simulink model "inv_im_param"  (R2026b)
settings: Solver=ode23tb  StopTime=param.sim.simlength  FixedStep=tc  MaxStep=param.glb_time.tc
values from neighbouring files (symbols this model uses):
  param = add_template_extras(param, options)    [init_model.m]
undefined symbols (not defined in the file or in its folder): magnitude
libraries: fl_lib x30, nesl_utility x13, lithium_ion_battery x1, induction_machine x1, dclink_with_center_tap x1, dead_time_generator_cmos_simulink x1, three_phase_pwm_modulator x1, three_phase_inverter_ideal_switch_based_model x1, three_phase_inverter_igbt_advanced_thermal_model x1, three_phase_inverter_mosfet_based_with_thermal_model x1, threephase_inductor_lib x1, simple_flexible_shaft x1
(part 2 of 3)

== system inv_im_param/inv_im_mod1/inverter/inverter/sv_pwm ==
  gate_cmds_uvw : Inport
  Bus Selector2 : BusSelector  OutputSignals=du(k),dv(k),dw(k)
  Constant1 : Constant  Value=param.inv.behav.pwm_phase_shift_mod1
  modulator1 : Subsystem
  td2tc_1 : TransferFcn  Denominator=[param.glb_time.tc 1]
  td2tc_2 : TransferFcn  Denominator=[param.glb_time.tc 1]
  td2tc_3 : TransferFcn  Denominator=[param.glb_time.tc 1]
  gate_cmds : Outport
  wires:
  modulator1/1(gate_cmds) -> gate_cmds/1
  Constant1/1 -> modulator1/4(phase)
  Bus Selector2/1 -> td2tc_1/1  "<du(k)>"
  Bus Selector2/2 -> td2tc_2/1  "<dv(k)>"
  Bus Selector2/3 -> td2tc_3/1  "<dw(k)>"
  gate_cmds_uvw/1 -> Bus Selector2/1
  td2tc_1/1 -> modulator1/1(u)  "du(t)"
  td2tc_3/1 -> modulator1/3(w)  "dw(t)"
  td2tc_2/1 -> modulator1/2(v)  "dv(t)"

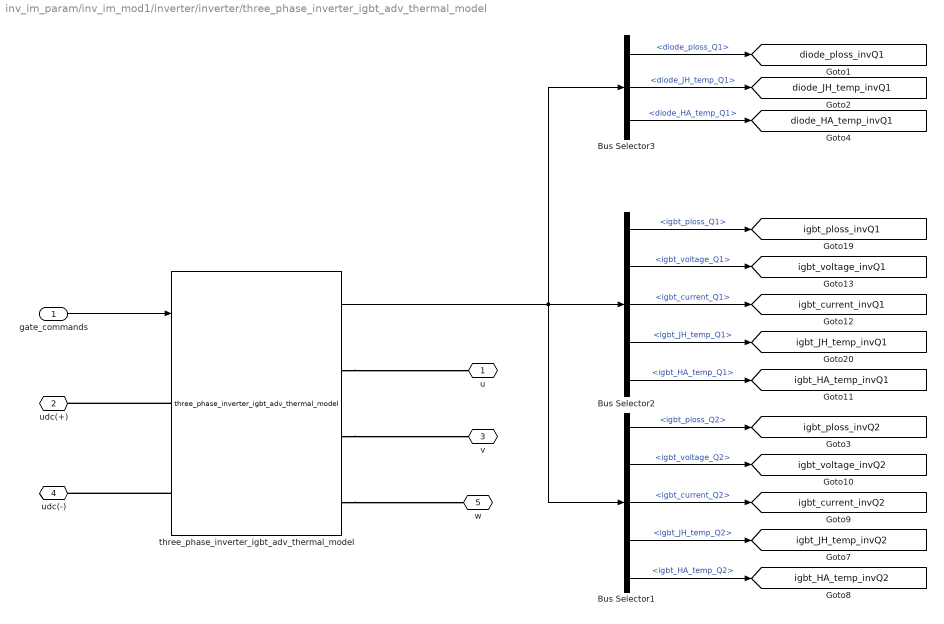
== system inv_im_param/inv_im_mod1/inverter/inverter/three_phase_inverter_igbt_adv_thermal_model ==
  gate_commands : Inport
  Bus Selector1 : BusSelector  OutputSignals=module_1.igbt_ploss_Q2,module_1.igbt_voltage_Q2,module_1.igbt_current_Q2,module_1.igbt_JH_temp_Q2,module_1.igbt_HA_temp_Q2
  Bus Selector2 : BusSelector  OutputSignals=module_1.igbt_ploss_Q1,module_1.igbt_voltage_Q1,module_1.igbt_current_Q1,module_1.igbt_JH_temp_Q1,module_1.igbt_HA_temp_Q1
  Bus Selector3 : BusSelector  OutputSignals=module_1.diode_ploss_Q1,module_1.diode_JH_temp_Q1,module_1.diode_HA_temp_Q1
  three_phase_inverter_igbt_adv_thermal_model : three_phase_inverter_igbt_advanced_thermal_model/three_phase_inverter_igbt_adv_thermal_model  mass_heatsink_m=param.thermal.weight  specific_heat_m=param.thermal.cp_al  rth_switch_HA_m=param.thermal.Rth_switch_HA  rth_switch_JH_m=param.inv.igbt.Rth_switch_JH  rth_diode_HA_m=param.thermal.Rth_diode_HA  rth_diode_JH_m=param.inv.igbt.Rth_diode_JH  Rce_on_m=param.inv.igbt.Rce_on  Vce_sat_m=param.inv.igbt.Vce_sat  Vth_m=param.inv.igbt.Vth  Eon_m=param.inv.igbt.Eon  Eoff_m=param.inv.igbt.Eoff  Erec_m=param.inv.igbt.Erec  Irr_m=param.inv.igbt.Irr  Voff_sw_loss_m=param.inv.igbt.Voff_sw_losses  Ion_sw_loss_m=param.inv.igbt.Ion_sw_losses  Vdon_diode_m=param.inv.igbt.Vdon_diode  Rdon_diode_m=param.inv.igbt.Rdon_diode  Csnubber_m=param.inv.igbt.Csnubber  Rsnubber_m=param.inv.igbt.Rsnubber  JunctionTermalMass_m=param.inv.igbt.JunctionTermalMass  Tambient_m=param.thermal.Tambient  DThs_init_m=param.thermal.DThs_init  Lstray_module_m=param.inv.igbt.Lstray_module  Cies_m=param.inv.igbt.Cies  tc_m=param.glb_time.tc
  u : PMIOPort  Side=Right
  udc(+) : PMIOPort  Port=2  Side=Left
  v : PMIOPort  Port=3  Side=Right
  udc(-) : PMIOPort  Port=4  Side=Left
  w : PMIOPort  Port=5  Side=Right
  tag scope: diode_HA_temp_invQ1=global, diode_JH_temp_invQ1=global, diode_ploss_invQ1=global, igbt_HA_temp_invQ1=global, igbt_HA_temp_invQ2=global, igbt_JH_temp_invQ1=global, igbt_JH_temp_invQ2=global, igbt_current_invQ1=global, igbt_current_invQ2=global, igbt_ploss_invQ1=global, igbt_ploss_invQ2=global, igbt_voltage_invQ1=global, igbt_voltage_invQ2=global
  wires:
  Bus Selector1/4 -> [igbt_JH_temp_invQ2]  "<igbt_JH_temp_Q2>"
  three_phase_inverter_igbt_adv_thermal_model/1 -> Bus Selector3/1, Bus Selector1/1, Bus Selector2/1
  Bus Selector1/2 -> [igbt_voltage_invQ2]  "<igbt_voltage_Q2>"
  Bus Selector1/3 -> [igbt_current_invQ2]  "<igbt_current_Q2>"
  Bus Selector1/5 -> [igbt_HA_temp_invQ2]  "<igbt_HA_temp_Q2>"
  Bus Selector2/2 -> [igbt_voltage_invQ1]  "<igbt_voltage_Q1>"
  Bus Selector2/1 -> [igbt_ploss_invQ1]  "<igbt_ploss_Q1>"
  Bus Selector2/3 -> [igbt_current_invQ1]  "<igbt_current_Q1>"
  Bus Selector1/1 -> [igbt_ploss_invQ2]  "<igbt_ploss_Q2>"
  gate_commands/1 -> three_phase_inverter_igbt_adv_thermal_model/1
  Bus Selector3/1 -> [diode_ploss_invQ1]  "<diode_ploss_Q1>"
  Bus Selector3/2 -> [diode_JH_temp_invQ1]  "<diode_JH_temp_Q1>"
  Bus Selector3/3 -> [diode_HA_temp_invQ1]  "<diode_HA_temp_Q1>"
  Bus Selector2/4 -> [igbt_JH_temp_invQ1]  "<igbt_JH_temp_Q1>"
  Bus Selector2/5 -> [igbt_HA_temp_invQ1]  "<igbt_HA_temp_Q1>"
  connections:
  three_phase_inverter_igbt_adv_thermal_model/LConn2 -- udc(-)/RConn1
  three_phase_inverter_igbt_adv_thermal_model/RConn1 -- u/RConn1
  three_phase_inverter_igbt_adv_thermal_model/RConn2 -- v/RConn1
  three_phase_inverter_igbt_adv_thermal_model/LConn1 -- udc(+)/RConn1
  three_phase_inverter_igbt_adv_thermal_model/RConn3 -- w/RConn1

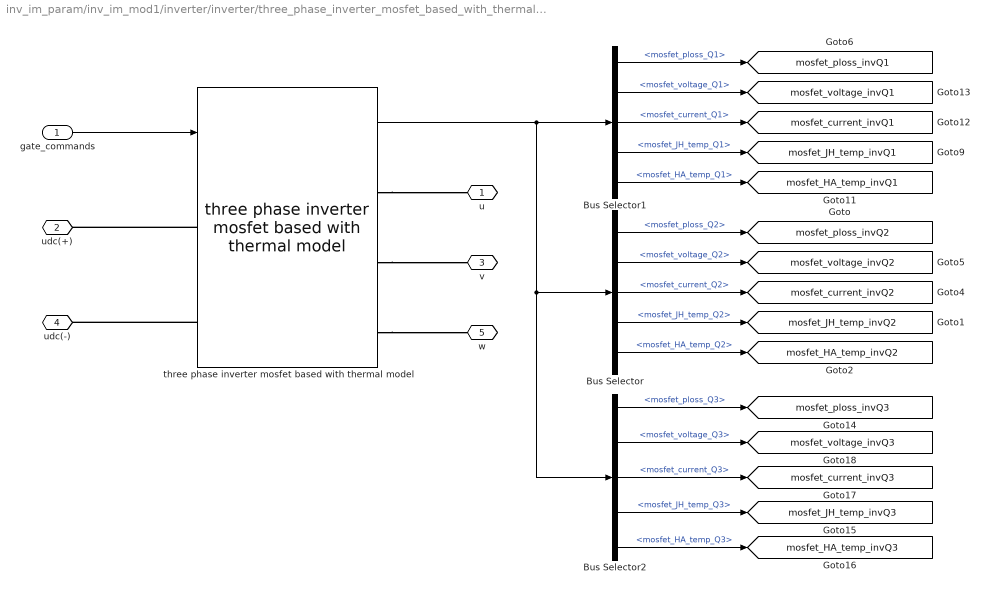
== system inv_im_param/inv_im_mod1/inverter/inverter/three_phase_inverter_mosfet_based_with_thermal_model ==
  gate_commands : Inport
  Bus Selector : BusSelector  OutputSignals=mosfet_ploss_Q2,mosfet_voltage_Q2,mosfet_current_Q2,mosfet_JH_temp_Q2,mosfet_HA_temp_Q2
  Bus Selector1 : BusSelector  OutputSignals=mosfet_ploss_Q1,mosfet_voltage_Q1,mosfet_current_Q1,mosfet_JH_temp_Q1,mosfet_HA_temp_Q1
  Bus Selector2 : BusSelector  OutputSignals=mosfet_ploss_Q3,mosfet_voltage_Q3,mosfet_current_Q3,mosfet_JH_temp_Q3,mosfet_HA_temp_Q3
  three phase inverter mosfet based with thermal model : three_phase_inverter_mosfet_based_with_thermal_model/three phase inverter mosfet based with thermal model  mass_heatsink_m=param.thermal.weight  specific_heat_m=param.thermal.cp_al  rth_mosfet_HA_m=param.thermal.Rth_diode_HA  rth_mosfet_JH_m=param.inv.mosfet.Rth_mosfet_JH  Rds_on_m=param.inv.mosfet.Rds_on  Vth_m=param.inv.mosfet.Vth  Eon_m=param.inv.mosfet.Eon  Eoff_m=param.inv.mosfet.Eoff  Voff_sw_loss_m=param.inv.mosfet.Voff_sw_losses  Ion_sw_loss_m=param.inv.mosfet.Ion_sw_losses  Vdon_diode_m=param.inv.mosfet.Vdon_diode  Rdon_diode_m=param.inv.mosfet.Rdon_diode  JunctionTermalMass_m=param.inv.mosfet.JunctionTermalMass  Tambient_m=param.thermal.Tambient  DThs_init_m=param.thermal.DThs_init
  u : PMIOPort  Side=Right
  udc(+) : PMIOPort  Port=2  Side=Left
  v : PMIOPort  Port=3  Side=Right
  udc(-) : PMIOPort  Port=4  Side=Left
  w : PMIOPort  Port=5  Side=Right
  tag scope: mosfet_HA_temp_invQ1=global, mosfet_HA_temp_invQ2=global, mosfet_HA_temp_invQ3=global, mosfet_JH_temp_invQ1=global, mosfet_JH_temp_invQ2=global, mosfet_JH_temp_invQ3=global, mosfet_current_invQ1=global, mosfet_current_invQ2=global, mosfet_current_invQ3=global, mosfet_ploss_invQ1=global, mosfet_ploss_invQ2=global, mosfet_ploss_invQ3=global, mosfet_voltage_invQ1=global, mosfet_voltage_invQ2=global, mosfet_voltage_invQ3=global
  wires:
  gate_commands/1 -> three phase inverter mosfet based with thermal model/1
  three phase inverter mosfet based with thermal model/1 -> Bus Selector/1, Bus Selector2/1, Bus Selector1/1
  Bus Selector2/1 -> [mosfet_ploss_invQ3]  "<mosfet_ploss_Q3>"
  Bus Selector2/2 -> [mosfet_voltage_invQ3]  "<mosfet_voltage_Q3>"
  Bus Selector2/3 -> [mosfet_current_invQ3]  "<mosfet_current_Q3>"
  Bus Selector2/5 -> [mosfet_HA_temp_invQ3]  "<mosfet_HA_temp_Q3>"
  Bus Selector2/4 -> [mosfet_JH_temp_invQ3]  "<mosfet_JH_temp_Q3>"
  Bus Selector/1 -> [mosfet_ploss_invQ2]  "<mosfet_ploss_Q2>"
  Bus Selector/2 -> [mosfet_voltage_invQ2]  "<mosfet_voltage_Q2>"
  Bus Selector/3 -> [mosfet_current_invQ2]  "<mosfet_current_Q2>"
  Bus Selector/4 -> [mosfet_JH_temp_invQ2]  "<mosfet_JH_temp_Q2>"
  Bus Selector/5 -> [mosfet_HA_temp_invQ2]  "<mosfet_HA_temp_Q2>"
  Bus Selector1/1 -> [mosfet_ploss_invQ1]  "<mosfet_ploss_Q1>"
  Bus Selector1/2 -> [mosfet_voltage_invQ1]  "<mosfet_voltage_Q1>"
  Bus Selector1/3 -> [mosfet_current_invQ1]  "<mosfet_current_Q1>"
  Bus Selector1/4 -> [mosfet_JH_temp_invQ1]  "<mosfet_JH_temp_Q1>"
  Bus Selector1/5 -> [mosfet_HA_temp_invQ1]  "<mosfet_HA_temp_Q1>"
  connections:
  three phase inverter mosfet based with thermal model/RConn3 -- w/RConn1
  three phase inverter mosfet based with thermal model/RConn2 -- v/RConn1
  three phase inverter mosfet based with thermal model/LConn1 -- udc(+)/RConn1
  three phase inverter mosfet based with thermal model/LConn2 -- udc(-)/RConn1
  three phase inverter mosfet based with thermal model/RConn1 -- u/RConn1

== system inv_im_param/inv_im_mod1/inverter_ctrl/im_control/Speed control ==
  rotor speed : Inport
  rotor speed ref : Inport  Port=2
  1/Ti : Gain  Gain=param.im.ctrl.kp_w  SaturateOnIntegerOverflow=on  OutDataTypeStr=Inherit: Same as input  ParamDataTypeStr=Inherit: Same as input
  Saturation : Saturate  UpperLimit=param.im.ctrl.iq_lim  LowerLimit=-param.im.ctrl.iq_lim
  Sum1 : Sum  Inputs=+++  SaturateOnIntegerOverflow=on
  Sum2 : Sum  Inputs=-+  SaturateOnIntegerOverflow=on
  Sum3 : Sum  Inputs=-+  SaturateOnIntegerOverflow=on
  Unit Delay4 : UnitDelay  SampleTime=-1
  kp : Gain  Gain=param.im.ctrl.ki_w*param.glb_time.ts_inv  SaturateOnIntegerOverflow=on  OutDataTypeStr=Inherit: Same as input  ParamDataTypeStr=Inherit: Same as input
  speed_tracking : Scope  NumInputPorts=3
      settings: ActiveDisplayYMinimum=-2.4020999013359527  ActiveDisplayYMaximum=1.8224555445928836  DataLoggingVariableName=ScopeData12
  torque_ref : Outport
  wires:
  1/Ti/1 -> Sum1/1, Sum3/1
  kp/1 -> Sum1/2
  Sum3/1 -> Unit Delay4/1
  Unit Delay4/1 -> Sum1/3
  rotor speed ref/1 -> speed_tracking/1, Sum2/2
  rotor speed/1 -> Sum2/1, speed_tracking/2
  Sum2/1 -> kp/1, 1/Ti/1
  Sum1/1 -> Saturation/1
  Saturation/1 -> torque_ref/1, speed_tracking/3, Sum3/2

== system inv_im_param/inv_im_mod1/inverter_ctrl/im_control/current_ctrl ==
  torque_ref : Inport
  Bus Creator1 : BusCreator  Inputs=2
  current_ctrl : Subsystem
  is uvw2xy : Subsystem
  rotor_flux_estimators : Subsystem
  us xy2alphabeta : Subsystem
  us xy2dq : Subsystem
  uvw2dq : Subsystem
  uab : Outport  VectorParamsAs1DForOutWhenUnconnected=off
  wires:
  [ubeta_pu_mod1] -> Bus Creator1/2  "u_ctrl_beta"
  [ualpha_pu_mod1] -> Bus Creator1/1  "u_ctrl_alpha"
  Bus Creator1/1 -> uab/1
  torque_ref/1 -> current_ctrl/1(iq_ref)  "torque_ref"
  [udcd_pu_inv_mod1] -> current_ctrl/2(udc_pu)

== system inv_im_param/inv_im_mod1/inverter_ctrl/im_control/encoder-sensorless-switch ==
  Step : Step  Time=param.im.mode.time_use_im_ekf  FinalValue=1 - param.im.mode.use_im_encoder
  Switch : Switch  Criteria=u2 > Threshold  Threshold=0.65  SaturateOnIntegerOverflow=off  InputSameDT=off
  Switch1 : Switch  Criteria=u2 > Threshold  Threshold=0.65  SaturateOnIntegerOverflow=off  InputSameDT=off
  double_integrator_observer : Subsystem
  tag scope: motor_phase_ctrl_mod1=scoped, motor_speed_pu_ctrl_mod1=scoped, phase_s=scoped, speed_pu_s=scoped
  wires:
  double_integrator_observer/1(phase_psm_hat) -> [motor_phase_ctrl_mod1]  "phase_psm_hat"
  double_integrator_observer/2(omega_pu_psm_hat) -> [motor_speed_pu_ctrl_mod1]  "omega_pu_psm_hat"
  [phased_im] -> double_integrator_observer/1(phase_psm)
  Step/1 -> Switch/2, Switch1/2
  [theta_s_mod1] -> Switch1/3
  [phase_elec_ekf_hat] -> Switch1/1
  [motor_speed_pu_ctrl_mod1] -> Switch/3
  [omega_elec_ekf_hat] -> Switch/1
  Switch/1 -> [speed_pu_s]
  Switch1/1 -> [phase_s]

== system inv_im_param/inv_im_mod1/inverter_ctrl/im_control/is inv quantizzation and one step delay ==
  is_abc_pu : Inport
  Demux : Demux  Outputs=3
  Mux : Mux  Inputs=3
  is inv quantizzation and one step delay : Subsystem
  isd_abc_pu : Outport
  wires:
  is inv quantizzation and one step delay/2(isd_v_pu) -> Mux/2
  is_abc_pu/1 -> Demux/1
  is inv quantizzation and one step delay/3(isd_w_pu) -> Mux/3
  is inv quantizzation and one step delay/1(isd_u_pu) -> Mux/1
  Demux/1 -> is inv quantizzation and one step delay/1(is_u_pu)
  Mux/1 -> isd_abc_pu/1
  Demux/3 -> is inv quantizzation and one step delay/3(is_w_pu)
  Demux/2 -> is inv quantizzation and one step delay/2(is_v_pu)

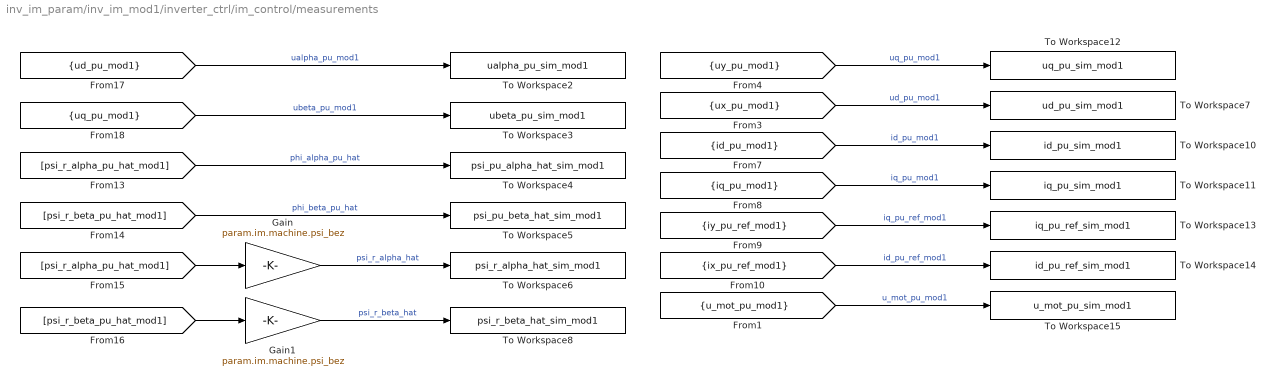
== system inv_im_param/inv_im_mod1/inverter_ctrl/im_control/measurements ==
  Gain : Gain  Gain=param.im.machine.psi_bez
  Gain1 : Gain  Gain=param.im.machine.psi_bez
  To Workspace10 : ToWorkspace  VariableName=id_pu_sim_mod1  SampleTime=-1
      settings: MaxDataPoints=param.glb_time.Ns_inv
  To Workspace11 : ToWorkspace  VariableName=iq_pu_sim_mod1  SampleTime=-1
      settings: MaxDataPoints=param.glb_time.Ns_inv
  To Workspace12 : ToWorkspace  VariableName=uq_pu_sim_mod1  SampleTime=-1
      settings: MaxDataPoints=param.glb_time.Ns_inv
  To Workspace13 : ToWorkspace  VariableName=iq_pu_ref_sim_mod1  SampleTime=-1
      settings: MaxDataPoints=param.glb_time.Ns_inv
  To Workspace14 : ToWorkspace  VariableName=id_pu_ref_sim_mod1  SampleTime=-1
      settings: MaxDataPoints=param.glb_time.Ns_inv
  To Workspace15 : ToWorkspace  VariableName=u_mot_pu_sim_mod1  SampleTime=-1
      settings: MaxDataPoints=param.glb_time.Ns_inv
  To Workspace2 : ToWorkspace  VariableName=ualpha_pu_sim_mod1  SampleTime=-1
      settings: MaxDataPoints=param.glb_time.Ns_inv
  To Workspace3 : ToWorkspace  VariableName=ubeta_pu_sim_mod1  SampleTime=-1
      settings: MaxDataPoints=param.glb_time.Ns_inv
  To Workspace4 : ToWorkspace  VariableName=psi_pu_alpha_hat_sim_mod1  SampleTime=-1
      settings: MaxDataPoints=param.glb_time.Ns_inv
  To Workspace5 : ToWorkspace  VariableName=psi_pu_beta_hat_sim_mod1  SampleTime=-1
      settings: MaxDataPoints=param.glb_time.Ns_inv
  To Workspace6 : ToWorkspace  VariableName=psi_r_alpha_hat_sim_mod1  SampleTime=-1
      settings: MaxDataPoints=param.glb_time.Ns_inv
  To Workspace7 : ToWorkspace  VariableName=ud_pu_sim_mod1  SampleTime=-1
      settings: MaxDataPoints=param.glb_time.Ns_inv
  To Workspace8 : ToWorkspace  VariableName=psi_r_beta_hat_sim_mod1  SampleTime=-1
      settings: MaxDataPoints=param.glb_time.Ns_inv
  wires:
  [psi_r_alpha_pu_hat_mod1] -> Gain/1
  [ud_pu_mod1] -> To Workspace2/1  "ualpha_pu_mod1"
  Gain/1 -> To Workspace6/1  "psi_r_alpha_hat"
  [psi_r_alpha_pu_hat_mod1] -> To Workspace4/1  "phi_alpha_pu_hat"
  [uq_pu_mod1] -> To Workspace3/1  "ubeta_pu_mod1"
  [psi_r_beta_pu_hat_mod1] -> To Workspace5/1  "phi_beta_pu_hat"
  Gain1/1 -> To Workspace8/1  "psi_r_beta_hat"
  [psi_r_beta_pu_hat_mod1] -> Gain1/1
  [u_mot_pu_mod1] -> To Workspace15/1  "u_mot_pu_mod1"
  [iy_pu_ref_mod1] -> To Workspace13/1  "iq_pu_ref_mod1"
  [ux_pu_mod1] -> To Workspace7/1  "ud_pu_mod1"
  [uy_pu_mod1] -> To Workspace12/1  "uq_pu_mod1"
  [iq_pu_mod1] -> To Workspace11/1  "iq_pu_mod1"
  [id_pu_mod1] -> To Workspace10/1  "id_pu_mod1"
  [ix_pu_ref_mod1] -> To Workspace14/1  "id_pu_ref_mod1"

== system inv_im_param/inv_im_mod1/inverter_ctrl/im_control/omega_pu ==
  Abs : Abs  SaturateOnIntegerOverflow=off
  flt : Subsystem
  abs(omega_pu) : Outport
  omega_pu : Outport  Port=2
  wires:
  Abs/1 -> flt/1(input)
  [speed_pu_s] -> Abs/1, omega_pu/1
  flt/1(output) -> abs(omega_pu)/1

== system inv_im_param/inv_im_mod1/inverter_ctrl/im_control/phase_acquisition ==
  phase_psm : Inport
  Quantizer : Quantizer  QuantizationInterval=param.meas.adc12_quantization
  Unit Delay : UnitDelay  SampleTime=-1
  Zero-Order Hold : ZeroOrderHold  SampleTime=-1
  phased_psm : Outport
  wires:
  Zero-Order Hold/1 -> Quantizer/1
  Unit Delay/1 -> phased_psm/1
  phase_psm/1 -> Zero-Order Hold/1
  Quantizer/1 -> Unit Delay/1

== system inv_im_param/inv_im_mod1/inverter_ctrl/im_control/phase_acquisition1 ==
  omega_psm : Inport
  Gain : Gain  Gain=1/param.im.machine.omega_bez
  Unit Delay : UnitDelay  SampleTime=-1
  Zero-Order Hold : ZeroOrderHold  SampleTime=-1
  omega_pu_psm : Outport
  wires:
  Zero-Order Hold/1 -> Gain/1
  omega_psm/1 -> Zero-Order Hold/1
  Unit Delay/1 -> omega_pu_psm/1
  Gain/1 -> Unit Delay/1

== system inv_im_param/inv_im_mod1/inverter_ctrl/im_control/phase_compensation_1 ==
  local_time : Inport
  master_time : Inport  Port=2
  Zero-Order Hold : ZeroOrderHold  SampleTime=-1
  Zero-Order Hold1 : ZeroOrderHold  SampleTime=-1
  alignment_ctrl : Subsystem
  y : Outport
  wires:
  local_time/1 -> Zero-Order Hold/1
  master_time/1 -> Zero-Order Hold1/1
  alignment_ctrl/1(dp) -> y/1
  Zero-Order Hold/1 -> alignment_ctrl/1(local_time)
  Zero-Order Hold1/1 -> alignment_ctrl/2(master_time)

== system inv_im_param/inv_im_mod1/inverter_ctrl/im_control/space_vector ==
  uab_out : Inport
  Bus Creator : BusCreator  Inputs=3
  Bus Selector : BusSelector  OutputSignals=da,db,dc
  Bus Selector1 : BusSelector  OutputSignals=u_ctrl_alpha,u_ctrl_beta
  C Caller : CCaller  FunctionName=sv_pwm_process_simulink  PortSpecificationStruct="%)30     .    V @   8    (     @         %    \"     4    !     0         %  0 \"0    $    _    07)G3F%M90  4&]R=$YA;64 4V-O<&4     26YD97@     5'EP90      4VEZ90      27-';&]B86P   X    P    !@    @    $          4    (     0    ,    !         !   P!O=70 #@   #     &    \"     0         !0    @    !     P    $         $  # &]U=  .    .     8    (    !          %    \"     $    &     0         0   ...(+2669 chars)"
  Constant : Constant  Value=param.glb_time.ts_inv
  Constant1 : Constant
  Data Type Conversion1 : DataTypeConversion  OutDataTypeStr=double  SaturateOnIntegerOverflow=off  RndMeth=Floor
  Data Type Conversion15 : DataTypeConversion  OutDataTypeStr=single  SaturateOnIntegerOverflow=off  RndMeth=Floor
  Data Type Conversion16 : DataTypeConversion  OutDataTypeStr=single  SaturateOnIntegerOverflow=off  RndMeth=Floor
  Data Type Conversion17 : DataTypeConversion  OutDataTypeStr=uint32  SaturateOnIntegerOverflow=off  RndMeth=Floor
  Data Type Conversion18 : DataTypeConversion  OutDataTypeStr=single  SaturateOnIntegerOverflow=off  RndMeth=Floor
  Data Type Conversion2 : DataTypeConversion  OutDataTypeStr=double  SaturateOnIntegerOverflow=off  RndMeth=Floor
  Data Type Conversion3 : DataTypeConversion  OutDataTypeStr=double  SaturateOnIntegerOverflow=off  RndMeth=Floor
  Gain1 : Gain  Gain=sqrt(3)/2
  Gain2 : Gain  Gain=sqrt(3)/2
  duvw : Outport
  wires:
  Data Type Conversion15/1 -> C Caller/2
  Bus Selector/2 -> Data Type Conversion2/1  "<db>"
  Data Type Conversion16/1 -> C Caller/3
  Data Type Conversion18/1 -> C Caller/1
  C Caller/1 -> Bus Selector/1
  Bus Creator/1 -> duvw/1
  Data Type Conversion17/1 -> C Caller/4
  Data Type Conversion1/1 -> Bus Creator/1  "du(k)"
  Bus Selector1/2 -> Gain2/1  "<u_ctrl_beta>"
  Bus Selector/3 -> Data Type Conversion3/1  "<dc>"
  Bus Selector1/1 -> Gain1/1  "<u_ctrl_alpha>"
  Data Type Conversion2/1 -> Bus Creator/2  "dv(k)"
  Gain2/1 -> Data Type Conversion15/1
  Bus Selector/1 -> Data Type Conversion1/1  "<da>"
  Gain1/1 -> Data Type Conversion18/1
  Data Type Conversion3/1 -> Bus Creator/3  "dw(k)"
  Constant/1 -> Data Type Conversion16/1
  uab_out/1 -> Bus Selector1/1
  Constant1/1 -> Data Type Conversion17/1

== system inv_im_param/inv_im_mod1/inverter_ctrl/im_control/speed_reference_generator ==
  Step : Step  Time=param.im.mode.time_start_motor_control
  Step1 : Step  Time=5  FinalValue=-2
  Sum : Sum  Inputs=|++
  flt : Subsystem
  omega_ref_pu : Outport
  tag scope: omega_ref_pu_mod1=scoped
  wires:
  Step/1 -> Sum/1
  Step1/1 -> Sum/2
  Sum/1 -> flt/1(input)
  flt/1(output) -> [omega_ref_pu_mod1], omega_ref_pu/1

== system inv_im_param/inv_im_mod1/inverter_ctrl/im_control/torque_reference ==
  rotor speed : Inport
  1-D Lookup Table : Lookup_n-D  NumberOfTableDimensions=1  BreakpointsForDimension1=param.load.rpm_base  Table=param.load.torque_base  InternalRulePriority=Speed  RndMeth=Simplest
  Gain : Gain  Gain=param.load.torque_overload_factor
  Gain1 : Gain  Gain=1/param.psm.machine.tau_bez
  Gain2 : Gain  Gain=param.psm.machine.rpm_nom
  Gain3 : Gain  Gain=-1
  Saturation : Saturate  UpperLimit=0  LowerLimit=-inf
  torque_ref : Outport
  wires:
  rotor speed/1 -> Gain2/1
  Saturation/1 -> torque_ref/1
  Gain1/1 -> Gain3/1
  1-D Lookup Table/1 -> Gain1/1
  Gain2/1 -> 1-D Lookup Table/1
  Gain/1 -> Saturation/1
  Gain3/1 -> Gain/1

== system inv_im_param/inv_im_mod1/inverter_ctrl/im_control/udc_acquisition ==
  udc_pu : Inport
  Quantizer : Quantizer  QuantizationInterval=param.meas.adc_quantization
  Unit Delay : UnitDelay  SampleTime=-1
  Zero-Order Hold : ZeroOrderHold  SampleTime=-1
  udcd_pu : Outport
  wires:
  Quantizer/1 -> Unit Delay/1
  udc_pu/1 -> Zero-Order Hold/1
  Unit Delay/1 -> udcd_pu/1
  Zero-Order Hold/1 -> Quantizer/1

== system inv_im_param/inv_im_mod1/inverter/inverter/sv_pwm/modulator1 ==
  u : Inport
  v : Inport  Port=2
  w : Inport  Port=3
  phase : Inport  Port=4
  Bus Creator : BusCreator  Inputs=3
  Three phase two level PWM generator with global TRGO : three_phase_pwm_modulator/Three phase two level PWM generator with global TRGO  f=param.glb_time.fPWM_INV  m_up=0.98  m_low=0.02  dead_time=0 %param.glb_time.dead_time_INV  pos_cmd_gate=15  neg_cmd_gate=-10  polarity=1  tc=param.glb_time.tc  double_sampling=param.glb_time.TRGO_INV_double_update
      link override gate commands/Bus Selector: OutputSignals=du(t)
      link override gate commands/Bus Selector1: OutputSignals=dv(t)
      link override gate commands/Bus Selector2: OutputSignals=dw(t)
  gate_cmds : Outport
  tag scope: TRGO_inv_module_1=global
  wires:
  [time_inv_module_1] -> Three phase two level PWM generator with global TRGO/1
  Bus Creator/1 -> Three phase two level PWM generator with global TRGO/3
  Three phase two level PWM generator with global TRGO/1 -> [TRGO_inv_module_1]
  u/1 -> Bus Creator/1
  v/1 -> Bus Creator/2
  w/1 -> Bus Creator/3
  phase/1 -> Three phase two level PWM generator with global TRGO/2
  Three phase two level PWM generator with global TRGO/2 -> gate_cmds/1

== system inv_im_param/inv_im_mod1/inverter_ctrl/im_control/current_ctrl/current_ctrl ==
  iq_ref : Inport
  udc_pu : Inport  Port=2
  Bus Creator : BusCreator  Inputs=2
  Bus Creator1 : BusCreator  Inputs=2
  Constant : Constant  Value=param.im.machine.psi_norm/param.im.machine.Lm_norm
  Sqrt : Sqrt
  Square : Math  Operator=square
  Square1 : Math  Operator=square
  Sum : Sum  Inputs=|++
  dq_pi_with_vector_antiwindup mod1 : Subsystem
  ix/iy tracking : Scope  NumInputPorts=2
      settings: ActiveDisplayYMinimum=0.23832511999512743  ActiveDisplayYMaximum=0.81515907316069991
  tag scope: ix_pu_ref_mod1=scoped, iy_pu_ref_mod1=scoped, u_mot_pu_mod1=scoped, ux_pu_mod1=scoped, uy_pu_mod1=scoped
  wires:
  [isy_pu_mod1] -> Bus Creator1/2, dq_pi_with_vector_antiwindup mod1/4(iq)  "isy_pu"
  [isx_pu_mod1] -> Bus Creator/2, dq_pi_with_vector_antiwindup mod1/2(id)  "isx_pu"
  iq_ref/1 -> [iy_pu_ref_mod1], Bus Creator1/1, dq_pi_with_vector_antiwindup mod1/3(iq_ref)  "isy_pu_ref"
  dq_pi_with_vector_antiwindup mod1/1(ctrl_d_u) -> [ux_pu_mod1], Square1/1
  dq_pi_with_vector_antiwindup mod1/2(ctrl_q_u) -> Square/1, [uy_pu_mod1]
  Square/1 -> Sum/1
  Sum/1 -> Sqrt/1
  Square1/1 -> Sum/2
  Sqrt/1 -> [u_mot_pu_mod1]
  Constant/1 -> [ix_pu_ref_mod1], Bus Creator/1, dq_pi_with_vector_antiwindup mod1/1(id_ref)  "isx_pu_ref"
  udc_pu/1 -> dq_pi_with_vector_antiwindup mod1/5(udc_pu)
  Bus Creator/1 -> ix/iy tracking/1
  Bus Creator1/1 -> ix/iy tracking/2

== system inv_im_param/inv_im_mod1/inverter_ctrl/im_control/current_ctrl/is uvw2xy ==
  Demux : Demux  Outputs=3
  alphabeta2dq : MATLAB Function  TreatAsAtomicUnit=on
  uvw2alphabeta : MATLAB Function  TreatAsAtomicUnit=on
  tag scope: isx_pu_mod1=scoped, isy_pu_mod1=scoped
  wires:
  [isd_uvw_inv_mod1] -> Demux/1
  Demux/1 -> uvw2alphabeta/1(u)  "iu"
  Demux/2 -> uvw2alphabeta/2(v)  "iv"
  Demux/3 -> uvw2alphabeta/3(w)  "iw"
  [phase_s] -> alphabeta2dq/3(gamma)
  uvw2alphabeta/1(alpha) -> alphabeta2dq/1(alpha)  "ialpha_pu"
  uvw2alphabeta/2(beta) -> alphabeta2dq/2(beta)  "ibeta_pu"
  alphabeta2dq/1(d) -> [isx_pu_mod1]  "isx_pu"
  alphabeta2dq/2(q) -> [isy_pu_mod1]  "isy_pu"

== system inv_im_param/inv_im_mod1/inverter_ctrl/im_control/current_ctrl/rotor_flux_estimators ==
  ekf : Subsystem
  sdl : Subsystem

== system inv_im_param/inv_im_mod1/inverter_ctrl/im_control/current_ctrl/us xy2alphabeta ==
  xy2dq : MATLAB Function  TreatAsAtomicUnit=on
  tag scope: ualpha_pu_mod1=scoped, ubeta_pu_mod1=scoped
  wires:
  xy2dq/2(beta) -> [ubeta_pu_mod1]
  xy2dq/1(alpha) -> [ualpha_pu_mod1]
  [uy_pu_mod1] -> xy2dq/2(q)
  [ux_pu_mod1] -> xy2dq/1(d)
  [phase_s] -> xy2dq/3(gamma)

== system inv_im_param/inv_im_mod1/inverter_ctrl/im_control/current_ctrl/us xy2dq ==
  xy2dq : MATLAB Function  TreatAsAtomicUnit=on
  tag scope: ud_pu_mod1=scoped, uq_pu_mod1=scoped
  wires:
  [ux_pu_mod1] -> xy2dq/1(d)
  [uy_pu_mod1] -> xy2dq/2(q)
  xy2dq/1(alpha) -> [ud_pu_mod1]
  xy2dq/2(beta) -> [uq_pu_mod1]
  [theta_slip_mod1] -> xy2dq/3(gamma)

== system inv_im_param/inv_im_mod1/inverter_ctrl/im_control/current_ctrl/uvw2dq ==
  Demux : Demux  Outputs=3
  alphabeta2dq : MATLAB Function  TreatAsAtomicUnit=on
  uvw2alphabeta : MATLAB Function  TreatAsAtomicUnit=on
  tag scope: ialpha_pu_mod1=scoped, ibeta_pu_mod1=scoped, id_pu_mod1=scoped, iq_pu_mod1=scoped
  wires:
  alphabeta2dq/2(q) -> [iq_pu_mod1]  "iq_pu"
  alphabeta2dq/1(d) -> [id_pu_mod1]  "id_pu"
  uvw2alphabeta/2(beta) -> alphabeta2dq/2(beta), [ibeta_pu_mod1]  "ibeta_pu"
  uvw2alphabeta/1(alpha) -> alphabeta2dq/1(alpha), [ialpha_pu_mod1]  "ialpha_pu"
  [motor_phase_ctrl_mod1] -> alphabeta2dq/3(gamma)
  Demux/3 -> uvw2alphabeta/3(w)  "iw"
  Demux/2 -> uvw2alphabeta/2(v)  "iv"
  Demux/1 -> uvw2alphabeta/1(u)  "iu"
  [isd_uvw_inv_mod1] -> Demux/1

== system inv_im_param/inv_im_mod1/inverter_ctrl/im_control/encoder-sensorless-switch/double_integrator_observer ==
  phase_psm : Inport
  Gain : Gain  Gain=param.im.ctrl.di_obs.komega
  Gain1 : Gain  Gain=param.im.ctrl.di_obs.ktheta
  Gain2 : Gain  Gain=param.im.machine.omega_bez
  Gain3 : Gain  Gain=1/param.im.machine.omega_bez
  Gain4 : Gain  Gain=param.glb_time.ts_inv
  Gain5 : Gain  Gain=param.glb_time.ts_inv
  Gain6 : Gain  Gain=param.glb_time.ts_inv
  Sum : Sum  Inputs=-+|
  Sum1 : Sum  Inputs=|++
  Sum2 : Sum  Inputs=|++
  Sum8 : Sum  Inputs=++|
  Unit Delay1 : UnitDelay  InitialCondition=pi  SampleTime=-1
  Unit Delay2 : UnitDelay  SampleTime=-1
  bounder1 : MATLAB Function  TreatAsAtomicUnit=on
  bounder2 : MATLAB Function  TreatAsAtomicUnit=on
  phase_psm_hat : Outport  VectorParamsAs1DForOutWhenUnconnected=off
  omega_pu_psm_hat : Outport  Port=2  VectorParamsAs1DForOutWhenUnconnected=off
  wires:
  Gain1/1 -> Gain6/1
  phase_psm/1 -> Sum/2
  Sum8/1 -> Unit Delay1/1
  Unit Delay1/1 -> bounder2/1(u)
  Sum1/1 -> Unit Delay2/1
  Gain/1 -> Gain4/1
  Unit Delay2/1 -> omega_pu_psm_hat/1, Sum1/2, Gain5/1
  Sum2/1 -> Sum8/2
  bounder2/1(y) -> Sum2/2, phase_psm_hat/1, Sum/1  "phase_hat"
  bounder1/1(y) -> Gain/1, Gain1/1
  Gain2/1 -> Sum8/1
  Gain3/1 -> Sum1/1
  Gain5/1 -> Gain2/1
  Sum/1 -> bounder1/1(u)
  Gain4/1 -> Gain3/1
  Gain6/1 -> Sum2/1

== system inv_im_param/inv_im_mod1/inverter_ctrl/im_control/is inv quantizzation and one step delay/is inv quantizzation and one step delay ==
  is_u_pu : Inport
  is_v_pu : Inport  Port=2
  is_w_pu : Inport  Port=3
  Gain3 : Gain  Gain=-1
  Gain4 : Gain  Gain=-1
  Gain5 : Gain  Gain=-1
  Quantizer : Quantizer  QuantizationInterval=param.meas.adc_quantization
  Quantizer1 : Quantizer  QuantizationInterval=param.meas.adc_quantization
  Quantizer2 : Quantizer  QuantizationInterval=param.meas.adc_quantization
  Unit Delay : UnitDelay  SampleTime=-1
  Unit Delay1 : UnitDelay  SampleTime=-1
  Unit Delay2 : UnitDelay  SampleTime=-1
  Zero-Order Hold : ZeroOrderHold  SampleTime=-1
  Zero-Order Hold1 : ZeroOrderHold  SampleTime=-1
  Zero-Order Hold2 : ZeroOrderHold  SampleTime=-1
  isd_u_pu : Outport
  isd_v_pu : Outport  Port=2
  isd_w_pu : Outport  Port=3
  wires:
  Unit Delay/1 -> Gain3/1
  Unit Delay1/1 -> Gain4/1
  Unit Delay2/1 -> Gain5/1
  Quantizer/1 -> Unit Delay/1
  Quantizer1/1 -> Unit Delay1/1
  Quantizer2/1 -> Unit Delay2/1
  is_u_pu/1 -> Zero-Order Hold/1
  is_v_pu/1 -> Zero-Order Hold1/1
  is_w_pu/1 -> Zero-Order Hold2/1
  Gain3/1 -> isd_u_pu/1
  Gain4/1 -> isd_v_pu/1
  Gain5/1 -> isd_w_pu/1
  Zero-Order Hold/1 -> Quantizer/1
  Zero-Order Hold1/1 -> Quantizer1/1
  Zero-Order Hold2/1 -> Quantizer2/1

== system inv_im_param/inv_im_mod1/inverter_ctrl/im_control/omega_pu/flt ==
  input : Inport
  Gain3 : Gain  Gain=param.ctrl.filters.inv.g1_161Hz
  Gain6 : Gain  Gain=param.ctrl.filters.inv.g0_161Hz
  Sum : Sum  Inputs=|++
  Unit Delay1 : UnitDelay  SampleTime=-1
  output : Outport  VectorParamsAs1DForOutWhenUnconnected=off
  wires:
  Gain6/1 -> Sum/1
  input/1 -> Gain6/1
  Unit Delay1/1 -> Gain3/1
  Gain3/1 -> Sum/2
  Sum/1 -> Unit Delay1/1, output/1

== system inv_im_param/inv_im_mod1/inverter_ctrl/im_control/phase_compensation_1/alignment_ctrl ==
  local_time : Inport
  master_time : Inport  Port=2
  Constant : Constant  Value=0
  Gain : Gain  Gain=-1
  Sum : Sum  Inputs=|+-
  pi : Subsystem  mask{kp=param.ctrl.kp_align, ki=param.ctrl.ki_align, lim_up=param.ctrl.lim_up_align, lim_down=param.ctrl.lim_down_align}
      mask prompts: ki "ki*ts"
      mask Display:
      | disp('pi()');
      | port_label('input', 1, 'u_ref');
      | port_label('input', 2, 'u');
      | port_label('output', 1, 'y');
  dp : Outport
  wires:
  master_time/1 -> Sum/1
  Sum/1 -> Gain/1
  Constant/1 -> pi/1(u_ref)
  local_time/1 -> Sum/2
  Gain/1 -> pi/2(u)
  pi/1(y) -> dp/1

== system inv_im_param/inv_im_mod1/inverter_ctrl/im_control/speed_reference_generator/flt ==
  input : Inport
  Gain3 : Gain  Gain=param.ctrl.filters.inv.g1_10Hz
  Gain6 : Gain  Gain=param.ctrl.filters.inv.g0_10Hz
  Sum : Sum  Inputs=|++
  Unit Delay1 : UnitDelay  SampleTime=-1
  output : Outport  VectorParamsAs1DForOutWhenUnconnected=off
  wires:
  Gain6/1 -> Sum/1
  input/1 -> Gain6/1
  Unit Delay1/1 -> Gain3/1
  Gain3/1 -> Sum/2
  Sum/1 -> Unit Delay1/1, output/1

== system inv_im_param/inv_im_mod1/inverter_ctrl/im_control/current_ctrl/current_ctrl/dq_pi_with_vector_antiwindup mod1 ==
  id_ref : Inport
  id : Inport  Port=2
  iq_ref : Inport  Port=3
  iq : Inport  Port=4
  udc_pu : Inport  Port=5
  Variant Source : VariantSource  VariantControls={param.im.impl.use_current_controller_from_simulink_module_1 == 1, param.im.impl.use_current_controller_from_ccaller_module_1 == 1}
  Variant Source1 : VariantSource  VariantControls={param.im.impl.use_current_controller_from_simulink_module_1 == 1, param.im.impl.use_current_controller_from_ccaller_module_1 == 1}
  dq_vector_pi : Subsystem
  dq_vector_pi_ccaller : Subsystem
  simulink/Ccaller VectorPI : Scope  NumInputPorts=2
      settings: ActiveDisplayYMinimum=-0.13069371384335679  ActiveDisplayYMaximum=1.1207013439270668
  ctrl_d_u : Outport
  ctrl_q_u : Outport  Port=2
  wires:
  id/1 -> dq_vector_pi_ccaller/1(id), dq_vector_pi/1(id)  "id"
  id_ref/1 -> dq_vector_pi_ccaller/2(id_ref), dq_vector_pi/2(id_ref)  "id_ref"
  iq/1 -> dq_vector_pi_ccaller/3(iq), dq_vector_pi/3(iq)  "iq"
  iq_ref/1 -> dq_vector_pi_ccaller/4(iq_ref), dq_vector_pi/4(iq_ref)  "iq_ref"
  dq_vector_pi/1(md_sat) -> Variant Source/1
  dq_vector_pi_ccaller/2(uq_ctrl_out) -> Variant Source1/2
  dq_vector_pi/2(mq_sat) -> Variant Source1/1
  dq_vector_pi_ccaller/1(ud_ctrl_out) -> Variant Source/2
  Variant Source/1 -> ctrl_d_u/1, simulink/Ccaller VectorPI/1  "ctrl_d_u"
  Variant Source1/1 -> simulink/Ccaller VectorPI/2, ctrl_q_u/1  "ctrl_q_u"
  udc_pu/1 -> dq_vector_pi_ccaller/5(udc_pu)

== system inv_im_param/inv_im_mod1/inverter_ctrl/im_control/current_ctrl/rotor_flux_estimators/ekf ==
  Bus Creator2 : BusCreator  Inputs=2
  Bus Creator3 : BusCreator  Inputs=2
  Gain : Gain  Gain=param.im.u_im_scale_ekf
  Gain1 : Gain  Gain=param.im.u_im_scale_ekf
  Mux : Mux  Inputs=2
  Mux1 : Mux  Inputs=2
  Terminator : Terminator
  Terminator1 : Terminator
  ekf/sdl : Scope  NumInputPorts=2
      settings: ActiveDisplayYMinimum=-3.9269903672129489  ActiveDisplayYMaximum=3.9269867690186091  DataLoggingVariableName=ScopeData13
  ekf/sdl1 : Scope  NumInputPorts=2
      settings: ActiveDisplayYMinimum=-3.9269903672129489  ActiveDisplayYMaximum=3.9269867690186091  DataLoggingVariableName=ScopeData19
  extended_kalman_observer : Subsystem  mask(IM extended Kalman filter){ts=param.im.ctrl.ekf.ts, omega_b=param.im.ctrl.ekf.omega_b, sigma_n=param.im.ctrl.ekf.sigma_n, rs_n=param.im.ctrl.ekf.rs_n, lm_n=param.im.ctrl.ekf.lm_n, lr_n=param.im.ctrl.ekf.lr_n, alpha_n=param.im.ctrl.ekf.alpha_n, kr=param.im.ctrl.ekf.kr, tau_m=param.im.ctrl.ekf.tau_m, q_diag=param.im.ctrl.ekf.q_diag, r_diag=param.im.ctrl.ekf.r_diag, p0_diag=param.im.ctrl.ekf.p0_diag, x0=param.im.ctrl.ekf.x0, n_hold=param.im.ctrl.ekf.n_hold, cov_order=param.im.ctrl.ekf.cov_order, n_delay_u=param.im.ctrl.ekf.n_delay_u}
      mask prompts: ts "ts: sampling time [s]"; omega_b "omega_b: base pulsation [rad/s]"; sigma_n "sigma_n: sigma*Ls of machine plus output inductor [pu]"; rs_n "rs_n: Rs of machine plus output inductor [pu]"; lm_n "lm_n: Lm [pu]"; lr_n "lr_n: Lr [pu]"; alpha_n "alpha_n: Rr/Lr [pu]"; kr "kr: Lm/Lr"; tau_m "tau_m: mechanical time constant [s]"; q_diag "q_diag: diagonal of Q per sample [pu^2]"; r_diag "r_diag: diagonal of R [pu^2]"; p0_diag "p0_diag: diagonal of P0 [pu^2]"; x0 "x0: initial state [pu]"; n_hold "n_hold: samples with speed and load torque held at zero"; cov_order "cov_order: order of the covariance transition matrix (1 or 2)"; n_delay_u "n_delay_u: delay of the voltage command [samples, >= 1]"
      mask help: Six-state extended Kalman filter of the induction machine, x = [i_alpha i_beta psi_alpha psi_beta omega T_load] in pu: rotor flux, its angle and the electrical speed from the voltage command and the measured current (algorithm ekf_im_step, data ekf_im_setup of the library). The voltage command is delayed by n_delay_u samples (2 in this model: current sampled one step late, command applied at the next PWM update) and multiplied by the measured DC-link voltage.
      mask Display:
      | disp('IM EKF');
      | port_label('input', 1, 'u_alpha_beta');
      | port_label('input', 2, 'i_alpha_beta');
      | port_label('input', 3, 'udc_pu');
      | port_label('output', 1, 'psi_alpha');
      | port_label('output', 2, 'psi_beta');
      | port_label('output', 3, 'theta');
      | port_label('output', 4, 'omega');
  tag scope: omega_elec_ekf_hat=scoped, phase_elec_ekf_hat=scoped
  wires:
  Mux/1 -> extended_kalman_observer/1(ualphabeta)
  Mux1/1 -> extended_kalman_observer/2(ialphabeta)
  [ialpha_pu_mod1] -> Mux1/1
  [ibeta_pu_mod1] -> Mux1/2
  extended_kalman_observer/3(phase_elec_ekf_hat) -> [phase_elec_ekf_hat], Bus Creator2/1  "phase_elec_ekf_hat"
  Gain/1 -> Mux/1  "um_alpha"
  Gain1/1 -> Mux/2  "um_beta"
  extended_kalman_observer/4(omega_elec_ekf_hat) -> [omega_elec_ekf_hat], Bus Creator3/1  "omega_elec_ekf_hat"
  Bus Creator2/1 -> ekf/sdl/1
  [theta_s_mod1] -> Bus Creator2/2  "phase_elec_sdl_hat"
  Bus Creator3/1 -> ekf/sdl/2
  [motor_speed_pu_ctrl_mod1] -> Bus Creator3/2  "motor_speed_pu_ctrl_mod1"
  [ualpha_pu_mod1] -> Gain/1
  [ubeta_pu_mod1] -> Gain1/1
  extended_kalman_observer/1(psi_alpha_ekf_hat) -> ekf/sdl1/1, Terminator/1
  extended_kalman_observer/2(psi_beta_ekf_hat) -> ekf/sdl1/2, Terminator1/1
  [udcd_pu_inv_mod1] -> extended_kalman_observer/3(udc_pu)  "udcd_pu_inv_mod1"

== system inv_im_param/inv_im_mod1/inverter_ctrl/im_control/current_ctrl/rotor_flux_estimators/sdl ==
  observer_from_rotor : Subsystem
  observer_performance_sdl : Scope  NumInputPorts=4
      settings: ActiveDisplayYMinimum=-1.8099572838063698  ActiveDisplayYMaximum=1.8361251727377448  DataLoggingVariableName=ScopeData15
  xy2dq : MATLAB Function  TreatAsAtomicUnit=on
  xy2dq1 : MATLAB Function  TreatAsAtomicUnit=on
  wires:
  [id_pu_mod1] -> xy2dq/1(d)
  [iq_pu_mod1] -> xy2dq/2(q)
  [motor_phase_ctrl_mod1] -> xy2dq1/3(gamma), xy2dq/3(gamma)
  [psi_r_d_hat_mod1] -> xy2dq1/1(d)
  [psi_r_q_hat_mod1] -> xy2dq1/2(q)
  xy2dq/1(alpha) -> observer_performance_sdl/1  "ialpha"
  xy2dq/2(beta) -> observer_performance_sdl/2  "ibeta"
  xy2dq1/1(alpha) -> observer_performance_sdl/3  "psi_alpha_hat_sdl"
  xy2dq1/2(beta) -> observer_performance_sdl/4  "psi_beta_hat_sdl"

== system inv_im_param/inv_im_mod1/inverter_ctrl/im_control/phase_compensation_1/alignment_ctrl/pi ==
  u_ref : Inport
  u : Inport  Port=2
  1/Ti : Gain  Gain=kp  SaturateOnIntegerOverflow=on  OutDataTypeStr=Inherit: Same as input  ParamDataTypeStr=Inherit: Same as input
  Saturation : Saturate  UpperLimit=lim_up  LowerLimit=lim_down
  Sum1 : Sum  Inputs=+++  SaturateOnIntegerOverflow=on
  Sum2 : Sum  Inputs=-+  SaturateOnIntegerOverflow=on
  Sum3 : Sum  Inputs=-+  SaturateOnIntegerOverflow=on
  Unit Delay4 : UnitDelay  SampleTime=-1
  kp : Gain  Gain=ki  SaturateOnIntegerOverflow=on  OutDataTypeStr=Inherit: Same as input  ParamDataTypeStr=Inherit: Same as input
  y : Outport
  wires:
  1/Ti/1 -> Sum1/1, Sum3/1
  kp/1 -> Sum1/2
  Sum3/1 -> Unit Delay4/1
  Unit Delay4/1 -> Sum1/3
  u_ref/1 -> Sum2/2
  u/1 -> Sum2/1
  Sum2/1 -> kp/1, 1/Ti/1
  Sum1/1 -> Saturation/1
  Saturation/1 -> Sum3/2, y/1

== system inv_im_param/inv_im_mod1/inverter_ctrl/im_control/current_ctrl/current_ctrl/dq_pi_with_vector_antiwindup mod1/dq_vector_pi ==
  id : Inport
  id_ref : Inport  Port=2
  iq : Inport  Port=3
  iq_ref : Inport  Port=4
  Sum1 : Sum  Inputs=|-+
  Sum2 : Sum  Inputs=|-+
  bounder1 : Subsystem
  bounder2 : Subsystem
  pi_d : Subsystem
  pi_q : Subsystem
  switch : Subsystem
  vector lenght : Subsystem
  md_sat : Outport
  mq_sat : Outport  Port=2
  wires:
  bounder2/2(clip) -> switch/2(clip 2)
  vector lenght/2(m) -> bounder1/3(m), bounder2/1(m)
  Sum2/1 -> pi_q/1(iq_tilde)
  pi_d/1(ud_out) -> vector lenght/1(md), bounder1/1(md)
  pi_q/1(Vqs_out) -> bounder2/3(mq), vector lenght/2(mq)
  vector lenght/1(m_1) -> bounder1/2(m_1), bounder2/2(m_1)
  switch/1(clip) -> pi_q/2(clip), pi_d/2(clip)
  iq/1 -> Sum2/1
  Sum1/1 -> pi_d/1(id_tilde)
  bounder1/2(clip) -> switch/1(clip 1)
  id/1 -> Sum1/1
  bounder1/1(md_sat) -> md_sat/1
  bounder2/1(mq_sat) -> mq_sat/1
  id_ref/1 -> Sum1/2
  iq_ref/1 -> Sum2/2
